simulink model "Y3Tiltrotor_sim3_IINDI_case2"  (R2025a)
settings: Solver=ode4  StartTime=0.0  StopTime=80  FixedStep=uavParam.sampleTime  RelTol=1e-3
PreLoadFcn:
  | filepath  = fileparts(get_param(bdroot, 'FileName'))
  | cd(filepath);
InitFcn:
  | Init_sim_IINDI_case2;
values from neighbouring files (symbols this model uses):
  a_HOD_p = 5    [Init_sim_IINDI_case2.m]    (also in Init_sim_IINDI_case2_1.m)
  a_HOD_q = 5    [Init_sim_IINDI_case2.m]    (also in Init_sim_IINDI_case2_1.m = 25)
  a_HOD_r = 5    [Init_sim_IINDI_case2.m]    (also in Init_sim_IINDI_case2_1.m)
  a_HOD_u = 5    [Init_sim_IINDI_case2.m]    (also in Init_sim_IINDI_case2_1.m = 15)
  a_HOD_v = 2    [Init_sim_IINDI_case2.m]    (also in Init_sim_IINDI_case2_1.m)
  a_HOD_w = 30    [Init_sim_IINDI_case2.m]    (also in Init_sim_IINDI_case2_1.m = 10)
  control = struct    [Init_sim_IINDI_case2.m]    (also in Init_sim_IINDI_case2_1.m)
  env = struct    [InitData.m]
  flightState = struct    [Init_sim_IINDI_case2.m]    (also in Init_sim_IINDI_case2_1.m)
  FWSpeed0 = 15    [Init_sim_IINDI_case2.m]    (also in Init_sim_IINDI_case2_1.m)
  k_lpf_p = 50    [Init_sim_IINDI_case2.m]    (also in Init_sim_IINDI_case2_1.m)
  k_lpf_q = 80    [Init_sim_IINDI_case2.m]    (also in Init_sim_IINDI_case2_1.m = 150)
  k_lpf_r = 100    [Init_sim_IINDI_case2.m]    (also in Init_sim_IINDI_case2_1.m)
  k_lpf_u = 8    [Init_sim_IINDI_case2.m]    (also in Init_sim_IINDI_case2_1.m)
  k_lpf_v = 1.5    [Init_sim_IINDI_case2.m]    (also in Init_sim_IINDI_case2_1.m)
  k_lpf_w = 50    [Init_sim_IINDI_case2.m]    (also in Init_sim_IINDI_case2_1.m)
  k_p = 5    [Init_sim_IINDI_case2.m]    (also in Init_sim_IINDI_case2_1.m)
  k_q = 12    [Init_sim_IINDI_case2.m]    (also in Init_sim_IINDI_case2_1.m)
  k_r = 0.1    [Init_sim_IINDI_case2.m]    (also in Init_sim_IINDI_case2_1.m)
  k_u = 0.2    [Init_sim_IINDI_case2.m]    (also in Init_sim_IINDI_case2_1.m = 1)
  k_v = 0.7    [Init_sim_IINDI_case2.m]    (also in Init_sim_IINDI_case2_1.m = 0.2)
  k_w = 2    [Init_sim_IINDI_case2.m]    (also in Init_sim_IINDI_case2_1.m)
  l_p = 30    [Init_sim_IINDI_case2.m]    (also in Init_sim_IINDI_case2_1.m)
  l_q = 15    [Init_sim_IINDI_case2.m]    (also in Init_sim_IINDI_case2_1.m)
  l_r = 25    [Init_sim_IINDI_case2.m]    (also in Init_sim_IINDI_case2_1.m)
  l_u = 1    [Init_sim_IINDI_case2.m]    (also in Init_sim_IINDI_case2_1.m = 0.8)
  l_v = 1.2    [Init_sim_IINDI_case2.m]    (also in Init_sim_IINDI_case2_1.m)
  l_w = 1    [Init_sim_IINDI_case2.m]    (also in Init_sim_IINDI_case2_1.m)
  lamda_p = 10    [Init_sim_IINDI_case2.m]    (also in Init_sim_IINDI_case2_1.m)
  lamda_q = 5    [Init_sim_IINDI_case2.m]    (also in Init_sim_IINDI_case2_1.m)
  lamda_r = 1    [Init_sim_IINDI_case2.m]    (also in Init_sim_IINDI_case2_1.m)
  lamda_u = 1    [Init_sim_IINDI_case2.m]    (also in Init_sim_IINDI_case2_1.m)
  lamda_v = 0.15    [Init_sim_IINDI_case2.m]    (also in Init_sim_IINDI_case2_1.m)
  lamda_w = 1    [Init_sim_IINDI_case2.m]    (also in Init_sim_IINDI_case2_1.m)
  uavParam = struct    [InitData.m]
undefined symbols (not defined in the file or in its folder): a_HOD, a_HOD_uvw, ControlSampleTime, F, Light, MIL, Newton, Raphson
libraries: slpidlib x30, SignalEditorBlockLib x15, simulink x3, aerolibtransform2 x3, sharedtransform x3, robotcorelib x3, matrix_library x3, aerolibasang x2, aerolibutil x2, aerolibwind2 x2, shared6dof x1, aerolibatmos2 x1
(part 6 of 7)

== system Y3Tiltrotor_sim3_IINDI_case2/Subsystem/多旋翼模态/Multirotor altitude control/Subsystem/Subsystem ==
  z_ref : Inport
  z : Inport  Port=2
  Action Port : ActionPort  ActionPortLabel=case [ 0 ]:
  Derivative : Derivative
  PID Controller : slpidlib/PID Controller  Controller=PID  Form=Parallel  TimeDomain=Continuous-time  UseExternalTs=off  SampleTime=ControlSampleTime  IntegratorMethod=Forward Euler  FilterMethod=Forward Euler  ControllerParametersSource=internal  P=control.MR.alt_P  I=control.MR.alt_I  UseKiTs=off  D=control.MR.alt_D  UseExternalDerivativeSource=off  N=100  UseFilter=on  TunerSelectOption=Transfer Function Based (PID Tuner App)  InitialConditionSource=internal  InitialConditionForIntegrator=0  InitialConditionForFilter=0  DifferentiatorICPrevScaledInput=0  ExternalReset=none  TrackingMode=off  Kt=1  LimitOutput=off  SatLimitsSource=internal  UpperSaturationLimit=control.maxMRvelocity  LowerSaturationLimit=-control.maxMRvelocity  LinearizeAsGain=on  AntiWindupMode=clamping  Kb=1  LimitIntegrator=off  UpperIntegratorSaturationLimit=inf  LowerIntegratorSaturationLimit=-inf  POutMin=[]  POutMax=[]  IOutMin=[]  IOutMax=[]  DOutMin=[]  DOutMax=[]  NOutMin=[]  NOutMax=[]  SumOutMin=[]  SumOutMax=[]  SaturationOutMin=[]  SaturationOutMax=[]  PParamMin=[]  PParamMax=[]  IParamMin=[]  IParamMax=[]  DParamMin=[]  DParamMax=[]  NParamMin=[]  NParamMax=[]  KbParamMin=[]  KbParamMax=[]  KtParamMin=[]  KtParamMax=[]  KbOutMin=[]  KbOutMax=[]  KtOutMin=[]  KtOutMax=[]  IntegratorOutMin=[]  IntegratorOutMax=[]  FilterOutMin=[]  FilterOutMax=[]  SumI1OutMin=[]  SumI1OutMax=[]  SumI2OutMin=[]  SumI2OutMax=[]  SumI3OutMin=[]  SumI3OutMax=[]  SumI4OutMin=[]  SumI4OutMax=[]  SumDOutMin=[]  SumDOutMax=[]  DifferentiatorOutMin=[]  DifferentiatorOutMax=[]  FilterDiffOutCoefMin=[]  FilterDiffOutCoefMax=[]  ReciprocalOutMin=[]  ReciprocalOutMax=[]  SumDenOutMin=[]  SumDenOutMax=[]  SumNumOutMin=[]  SumNumOutMax=[]  DivideOutMin=[]  DivideOutMax=[]  UdiffTsProdOutMin=[]  UdiffTsProdOutMax=[]  NTsProdOutMin=[]  NTsProdOutMax=[]  UintegralTsProdOutMin=[]  UintegralTsProdOutMax=[]  UngainTsProdOutMin=[]  UngainTsProdOutMax=[]  ClampingZeroOutDataTypeStr=Inherit: Inherit via back propagation  ClampingZeroOutMin=[]  ClampingZeroOutMax=[]  FilterDenConstantOutDataTypeStr=Inherit: Inherit via back propagation  FilterDenConstantOutMin=[]  FilterDenConstantOutMax=[]  PCopyOutDataTypeStr=Inherit: Inherit via back propagation  PCopyOutMin=[]  PCopyOutMax=[]  NCopyOutDataTypeStr=Inherit: Inherit via back propagation  NCopyOutMin=[]  NCopyOutMax=[]  IntegratorContinuousStateAttributes=''  IntegratorStateMustResolveToSignalObject=off  IntegratorRTWStateStorageClass=Auto  FilterContinuousStateAttributes=''  FilterStateMustResolveToSignalObject=off  FilterRTWStateStorageClass=Auto  ParallelPVariant=InternalParameters  IdealPVariant=Disabled  IVariant=InternalParameters  DVariant=InternalParameters  IntegratorVariant=Continuous  SatVariant=Disabled  AWVariant=Passthrough  PCopyVariant=Disabled  TRVariant=Disabled  FdbkBlocksVariant=Forward  IdealPFdbkVariant=Disabled  SatFdbkVariant=Disabled  DerivativeFilterVariant=ContFilter  NVariant=InternalParameters  NCopyVariant=Disabled  FilterICVariant=InternalICsFilter  IntegratorICVariant=InternalICs  ExternalResetVariant=Disabled  TRSumVariant=Passthrough  SumFdbkVariant=Disabled  SumVariant=Sum_PID  TsampFilterVariant=InternalTs  TsampNgainVariant=Passthrough  TsampIntegralVariant=Disabled_SignalSpec  ExternalSaturationOutDataTypeStr=Inherit: Same as second input  DerivativeSourceVariant=ErrorSignal  PreIntVariant=InternalPreInt
  Saturation : Saturate  UpperLimit=control.maxMRvelocity  LowerLimit=-control.maxMRvelocity
  Sum : Sum  Inputs=|+-
  Sum1 : Sum  Inputs=++|
  Transfer Fcn1 : TransferFcn  Numerator=[5]  Denominator=[1 5]
  Transfer Fcn7 : TransferFcn  Numerator=[10]  Denominator=[1 10]
  PID_vz_cmd : Outport
  wires:
  z_ref/1 -> Transfer Fcn1/1
  z/1 -> Sum/2
  Sum/1 -> PID Controller/1  "e_z_IINDI"
  PID Controller/1 -> Sum1/2
  Derivative/1 -> Transfer Fcn7/1
  Sum1/1 -> Saturation/1
  Saturation/1 -> PID_vz_cmd/1
  Transfer Fcn7/1 -> Sum1/1
  Transfer Fcn1/1 -> Derivative/1, Sum/1  "z_ref"

== system Y3Tiltrotor_sim3_IINDI_case2/Subsystem/多旋翼模态/Multirotor attitude control (IINDI)/INDI in vector form/Subsystem ==
  original : Inport
  Demux : Demux  Outputs=3
  Mux : Mux  Inputs=3
  Transfer Fcn1 : TransferFcn  Numerator=[k_lpf_q]  Denominator=[1 k_lpf_q]
  Transfer Fcn2 : TransferFcn  Numerator=[k_lpf_r]  Denominator=[1 k_lpf_r]
  Transfer Fcn3 : TransferFcn  Numerator=[k_lpf_p]  Denominator=[1 k_lpf_p]
  LPF : Outport
  wires:
  Demux/2 -> Transfer Fcn1/1
  Demux/1 -> Transfer Fcn3/1
  Mux/1 -> LPF/1
  Transfer Fcn3/1 -> Mux/1
  Transfer Fcn1/1 -> Mux/2
  Transfer Fcn2/1 -> Mux/3
  Demux/3 -> Transfer Fcn2/1
  original/1 -> Demux/1

== system Y3Tiltrotor_sim3_IINDI_case2/Subsystem/多旋翼模态/Multirotor attitude control (IINDI)/INDI in vector form/Subsystem1 ==
  original : Inport
  Demux : Demux  Outputs=3
  Mux : Mux  Inputs=3
  Transfer Fcn1 : TransferFcn  Numerator=[k_lpf_q]  Denominator=[1 k_lpf_q]
  Transfer Fcn2 : TransferFcn  Numerator=[k_lpf_r]  Denominator=[1 k_lpf_r]
  Transfer Fcn3 : TransferFcn  Numerator=[k_lpf_p]  Denominator=[1 k_lpf_p]
  LPF : Outport
  wires:
  Demux/2 -> Transfer Fcn1/1
  Demux/1 -> Transfer Fcn3/1
  Mux/1 -> LPF/1
  Transfer Fcn3/1 -> Mux/1
  Transfer Fcn1/1 -> Mux/2
  Transfer Fcn2/1 -> Mux/3
  Demux/3 -> Transfer Fcn2/1
  original/1 -> Demux/1

== system Y3Tiltrotor_sim3_IINDI_case2/Subsystem/多旋翼模态/Multirotor attitude control (IINDI)/INDI in vector form/Subsystem2 ==
  original : Inport
  Demux : Demux  Outputs=3
  Mux : Mux  Inputs=3
  Transfer Fcn1 : TransferFcn  Numerator=[k_lpf_q]  Denominator=[1 k_lpf_q]
  Transfer Fcn2 : TransferFcn  Numerator=[k_lpf_r]  Denominator=[1 k_lpf_r]
  Transfer Fcn3 : TransferFcn  Numerator=[k_lpf_p]  Denominator=[1 k_lpf_p]
  LPF : Outport
  wires:
  Demux/2 -> Transfer Fcn1/1
  Demux/1 -> Transfer Fcn3/1
  Mux/1 -> LPF/1
  Transfer Fcn3/1 -> Mux/1
  Transfer Fcn1/1 -> Mux/2
  Transfer Fcn2/1 -> Mux/3
  Demux/3 -> Transfer Fcn2/1
  original/1 -> Demux/1

== system Y3Tiltrotor_sim3_IINDI_case2/Subsystem/多旋翼模态/Multirotor attitude control (IINDI)/Improved INDI in vector form/6阶HOD ==
  X1 : Inport
  Gain : Gain  Gain=[4*a_HOD_p^2 0 0;0 4*a_HOD_q^2 0;0 0 4*a_HOD_r^2]  Multiplication=Matrix(K*u) (u vector)
  Gain1 : Gain  Gain=[4*a_HOD_p 0 0;0 4*a_HOD_q 0;0 0 4*a_HOD_r]  Multiplication=Matrix(K*u) (u vector)
  Integrator : Integrator  InitialCondition=[0 0 0]'
  Integrator1 : Integrator  InitialCondition=[0 0 0]'
  Sum : Sum  Inputs=|+-
  Sum1 : Sum  Inputs=++|
  X1_dot_hat : Outport
  wires:
  Gain1/1 -> Sum1/1
  Integrator1/1 -> Sum1/2  "x2_hat"
  Gain/1 -> Integrator1/1
  Sum1/1 -> Integrator/1, X1_dot_hat/1
  Sum/1 -> Gain1/1, Gain/1
  X1/1 -> Sum/1
  Integrator/1 -> Sum/2  "x1_hat"

== system Y3Tiltrotor_sim3_IINDI_case2/Subsystem/多旋翼模态/Multirotor attitude control (IINDI)/Improved INDI in vector form/6阶HOD1 ==
  X1 : Inport
  Gain : Gain  Gain=[4*a_HOD_p^2 0 0;0 4*a_HOD_q^2 0;0 0 4*a_HOD_r^2]  Multiplication=Matrix(K*u) (u vector)
  Gain1 : Gain  Gain=[4*a_HOD_p 0 0;0 4*a_HOD_q 0;0 0 4*a_HOD_r]  Multiplication=Matrix(K*u) (u vector)
  Integrator : Integrator  InitialCondition=[0 0 0]'
  Integrator1 : Integrator  InitialCondition=[0 0 0]'
  Sum : Sum  Inputs=|+-
  Sum1 : Sum  Inputs=++|
  X1_dot_hat : Outport
  wires:
  Integrator/1 -> Sum/2  "x1_hat"
  X1/1 -> Sum/1
  Sum/1 -> Gain/1, Gain1/1
  Sum1/1 -> X1_dot_hat/1, Integrator/1
  Gain/1 -> Integrator1/1
  Integrator1/1 -> Sum1/2  "x2_hat"
  Gain1/1 -> Sum1/1

== system Y3Tiltrotor_sim3_IINDI_case2/Subsystem/多旋翼模态/Multirotor attitude control (IINDI)/Improved INDI in vector form/CFO ==
  x1_dot : Inport
  x1 : Inport  Port=2
  bu : Inport  Port=3
  Gain : Gain  Gain=[l_p 0 0;0 l_q 0;0 0 l_r]  Multiplication=Matrix(K*u) (u vector)
  Gain1 : Gain  Gain=[lamda_p 0 0;0 lamda_q 0;0 0 lamda_r]  Multiplication=Matrix(K*u) (u vector)
  Integrator : Integrator  InitialCondition=[0 0 0]'
  Integrator1 : Integrator  InitialCondition=[0 0 0]'
  Sum : Sum  Inputs=|+-
  Sum1 : Sum  Inputs=+++
  Sum2 : Sum  Inputs=++|
  d_hat : Outport
  wires:
  Sum2/1 -> d_hat/1, Sum1/1
  Integrator1/1 -> Sum2/2  "x2_hat"
  Gain1/1 -> Integrator1/1
  Sum/1 -> Gain/1
  Gain/1 -> Gain1/1, Sum2/1
  bu/1 -> Sum1/3
  x1_dot/1 -> Sum1/2
  Sum1/1 -> Integrator/1
  Integrator/1 -> Sum/2  "x1_hat"
  x1/1 -> Sum/1

== system Y3Tiltrotor_sim3_IINDI_case2/Subsystem/多旋翼模态/Multirotor attitude control (IINDI)/Improved INDI in vector form/Subsystem ==
  original : Inport
  Demux : Demux  Outputs=3
  Mux : Mux  Inputs=3
  Transfer Fcn1 : TransferFcn  Numerator=[k_lpf_q]  Denominator=[1 k_lpf_q]
  Transfer Fcn2 : TransferFcn  Numerator=[k_lpf_r]  Denominator=[1 k_lpf_r]
  Transfer Fcn3 : TransferFcn  Numerator=[k_lpf_p]  Denominator=[1 k_lpf_p]
  LPF : Outport
  wires:
  Demux/2 -> Transfer Fcn1/1
  Demux/1 -> Transfer Fcn3/1
  Mux/1 -> LPF/1
  Transfer Fcn3/1 -> Mux/1
  Transfer Fcn1/1 -> Mux/2
  Transfer Fcn2/1 -> Mux/3
  Demux/3 -> Transfer Fcn2/1
  original/1 -> Demux/1

== system Y3Tiltrotor_sim3_IINDI_case2/Subsystem/多旋翼模态/Multirotor attitude control (IINDI)/Improved INDI in vector form/Subsystem2 ==
  original : Inport
  Demux : Demux  Outputs=3
  Mux : Mux  Inputs=3
  Transfer Fcn1 : TransferFcn  Numerator=[k_lpf_q]  Denominator=[1 k_lpf_q]
  Transfer Fcn2 : TransferFcn  Numerator=[k_lpf_r]  Denominator=[1 k_lpf_r]
  Transfer Fcn3 : TransferFcn  Numerator=[k_lpf_p]  Denominator=[1 k_lpf_p]
  LPF : Outport
  wires:
  Demux/2 -> Transfer Fcn1/1
  Demux/1 -> Transfer Fcn3/1
  Mux/1 -> LPF/1
  Transfer Fcn3/1 -> Mux/1
  Transfer Fcn1/1 -> Mux/2
  Transfer Fcn2/1 -> Mux/3
  Demux/3 -> Transfer Fcn2/1
  original/1 -> Demux/1

== system Y3Tiltrotor_sim3_IINDI_case2/Subsystem/多旋翼模态/Multirotor attitude control (IINDI)/Improved INDI_p/2阶HOD ==
  X1 : Inport
  Gain : Gain  Gain=4*a_HOD^2
  Gain1 : Gain  Gain=4*a_HOD
  Integrator : Integrator
  Integrator1 : Integrator
  Sum : Sum  Inputs=|+-
  Sum1 : Sum  Inputs=++|
  X1_dot_hat : Outport
  wires:
  Gain1/1 -> Sum1/1
  Integrator1/1 -> Sum1/2  "x2_hat"
  Gain/1 -> Integrator1/1
  Sum1/1 -> Integrator/1, X1_dot_hat/1
  Sum/1 -> Gain1/1, Gain/1
  X1/1 -> Sum/1
  Integrator/1 -> Sum/2  "x1_hat"

== system Y3Tiltrotor_sim3_IINDI_case2/Subsystem/多旋翼模态/Multirotor attitude control (IINDI)/Improved INDI_p/CFO ==
  x1_dot : Inport
  x1 : Inport  Port=2
  bu : Inport  Port=3
  Gain : Gain  Gain=l_p
  Gain1 : Gain  Gain=lamda_p
  Integrator : Integrator
  Integrator1 : Integrator
  Sum : Sum  Inputs=|+-
  Sum1 : Sum  Inputs=+++
  Sum2 : Sum  Inputs=++|
  d_hat : Outport
  wires:
  Sum2/1 -> d_hat/1, Sum1/1
  Integrator1/1 -> Sum2/2  "x2_hat"
  Gain1/1 -> Integrator1/1
  Sum/1 -> Gain/1
  Gain/1 -> Gain1/1, Sum2/1
  bu/1 -> Sum1/3
  x1_dot/1 -> Sum1/2
  Sum1/1 -> Integrator/1
  Integrator/1 -> Sum/2  "x1_hat"
  x1/1 -> Sum/1

== system Y3Tiltrotor_sim3_IINDI_case2/Subsystem/多旋翼模态/Multirotor attitude control (IINDI)/Improved INDI_q/2阶HOD ==
  X1 : Inport
  Gain : Gain  Gain=4*a_HOD^2
  Gain1 : Gain  Gain=4*a_HOD
  Integrator : Integrator
  Integrator1 : Integrator
  Sum : Sum  Inputs=|+-
  Sum1 : Sum  Inputs=++|
  X1_dot_hat : Outport
  wires:
  Integrator/1 -> Sum/2  "x1_hat"
  X1/1 -> Sum/1
  Sum/1 -> Gain/1, Gain1/1
  Sum1/1 -> X1_dot_hat/1, Integrator/1
  Gain/1 -> Integrator1/1
  Integrator1/1 -> Sum1/2  "x2_hat"
  Gain1/1 -> Sum1/1

== system Y3Tiltrotor_sim3_IINDI_case2/Subsystem/多旋翼模态/Multirotor attitude control (IINDI)/Improved INDI_q/CFO ==
  x1_dot : Inport
  x1 : Inport  Port=2
  bu : Inport  Port=3
  Gain : Gain  Gain=l_q
  Gain1 : Gain  Gain=lamda_q
  Integrator : Integrator
  Integrator1 : Integrator
  Sum : Sum  Inputs=|+-
  Sum1 : Sum  Inputs=+++
  Sum2 : Sum  Inputs=++|
  d_hat : Outport
  wires:
  x1/1 -> Sum/1
  Integrator/1 -> Sum/2  "x1_hat"
  Sum1/1 -> Integrator/1
  x1_dot/1 -> Sum1/2
  bu/1 -> Sum1/3
  Gain/1 -> Sum2/1, Gain1/1
  Sum/1 -> Gain/1
  Gain1/1 -> Integrator1/1
  Integrator1/1 -> Sum2/2  "x2_hat"
  Sum2/1 -> Sum1/1, d_hat/1

== system Y3Tiltrotor_sim3_IINDI_case2/Subsystem/多旋翼模态/Multirotor attitude control (IINDI)/Improved INDI_r/2阶HOD ==
  X1 : Inport
  Gain : Gain  Gain=4*a_HOD^2
  Gain1 : Gain  Gain=4*a_HOD
  Integrator : Integrator
  Integrator1 : Integrator
  Sum : Sum  Inputs=|+-
  Sum1 : Sum  Inputs=++|
  X1_dot_hat : Outport
  wires:
  Gain1/1 -> Sum1/1
  Integrator1/1 -> Sum1/2  "x2_hat"
  Gain/1 -> Integrator1/1
  Sum1/1 -> Integrator/1, X1_dot_hat/1
  Sum/1 -> Gain1/1, Gain/1
  X1/1 -> Sum/1
  Integrator/1 -> Sum/2  "x1_hat"

== system Y3Tiltrotor_sim3_IINDI_case2/Subsystem/多旋翼模态/Multirotor attitude control (IINDI)/Improved INDI_r/CFO ==
  x1_dot : Inport
  x1 : Inport  Port=2
  bu : Inport  Port=3
  Gain : Gain  Gain=l_r
  Gain1 : Gain  Gain=lamda_r
  Integrator : Integrator
  Integrator1 : Integrator
  Sum : Sum  Inputs=|+-
  Sum1 : Sum  Inputs=+++
  Sum2 : Sum  Inputs=++|
  d_hat : Outport
  wires:
  Sum2/1 -> d_hat/1, Sum1/1
  Integrator1/1 -> Sum2/2  "x2_hat"
  Gain1/1 -> Integrator1/1
  Sum/1 -> Gain/1
  Gain/1 -> Gain1/1, Sum2/1
  bu/1 -> Sum1/3
  x1_dot/1 -> Sum1/2
  Sum1/1 -> Integrator/1
  Integrator/1 -> Sum/2  "x1_hat"
  x1/1 -> Sum/1

== system Y3Tiltrotor_sim3_IINDI_case2/Subsystem/多旋翼模态/Multirotor attitude control (IINDI)/Subsystem/Subsystem ==
  Euler_d : Inport
  Euler : Inport  Port=2
  Action Port : ActionPort  ActionPortLabel=case [ 0 ]:
  Gain1 : Gain  Gain=pi/180
  PID Controller4 : slpidlib/PID Controller  Controller=PI  Form=Parallel  TimeDomain=Continuous-time  UseExternalTs=off  SampleTime=ControlSampleTime  IntegratorMethod=Forward Euler  FilterMethod=Forward Euler  ControllerParametersSource=internal  P=control.MR.yaw_P  I=control.MR.yaw_I  UseKiTs=off  D=0  UseExternalDerivativeSource=off  N=100  UseFilter=on  TunerSelectOption=Transfer Function Based (PID Tuner App)  InitialConditionSource=internal  InitialConditionForIntegrator=0  InitialConditionForFilter=0  DifferentiatorICPrevScaledInput=0  ExternalReset=none  TrackingMode=off  Kt=1  LimitOutput=on  SatLimitsSource=internal  UpperSaturationLimit=control.maxRollRate  LowerSaturationLimit=control.minRollRate  LinearizeAsGain=on  AntiWindupMode=clamping  Kb=1  LimitIntegrator=off  UpperIntegratorSaturationLimit=inf  LowerIntegratorSaturationLimit=-inf  POutMin=[]  POutMax=[]  IOutMin=[]  IOutMax=[]  DOutMin=[]  DOutMax=[]  NOutMin=[]  NOutMax=[]  SumOutMin=[]  SumOutMax=[]  SaturationOutMin=[]  SaturationOutMax=[]  PParamMin=[]  PParamMax=[]  IParamMin=[]  IParamMax=[]  DParamMin=[]  DParamMax=[]  NParamMin=[]  NParamMax=[]  KbParamMin=[]  KbParamMax=[]  KtParamMin=[]  KtParamMax=[]  KbOutMin=[]  KbOutMax=[]  KtOutMin=[]  KtOutMax=[]  IntegratorOutMin=[]  IntegratorOutMax=[]  FilterOutMin=[]  FilterOutMax=[]  SumI1OutMin=[]  SumI1OutMax=[]  SumI2OutMin=[]  SumI2OutMax=[]  SumI3OutMin=[]  SumI3OutMax=[]  SumI4OutMin=[]  SumI4OutMax=[]  SumDOutMin=[]  SumDOutMax=[]  DifferentiatorOutMin=[]  DifferentiatorOutMax=[]  FilterDiffOutCoefMin=[]  FilterDiffOutCoefMax=[]  ReciprocalOutMin=[]  ReciprocalOutMax=[]  SumDenOutMin=[]  SumDenOutMax=[]  SumNumOutMin=[]  SumNumOutMax=[]  DivideOutMin=[]  DivideOutMax=[]  UdiffTsProdOutMin=[]  UdiffTsProdOutMax=[]  NTsProdOutMin=[]  NTsProdOutMax=[]  UintegralTsProdOutMin=[]  UintegralTsProdOutMax=[]  UngainTsProdOutMin=[]  UngainTsProdOutMax=[]  ClampingZeroOutDataTypeStr=Inherit: Inherit via back propagation  ClampingZeroOutMin=[]  ClampingZeroOutMax=[]  FilterDenConstantOutDataTypeStr=Inherit: Inherit via back propagation  FilterDenConstantOutMin=[]  FilterDenConstantOutMax=[]  PCopyOutDataTypeStr=Inherit: Inherit via back propagation  PCopyOutMin=[]  PCopyOutMax=[]  NCopyOutDataTypeStr=Inherit: Inherit via back propagation  NCopyOutMin=[]  NCopyOutMax=[]  IntegratorContinuousStateAttributes=''  IntegratorStateMustResolveToSignalObject=off  IntegratorRTWStateStorageClass=Auto  FilterContinuousStateAttributes=''  FilterStateMustResolveToSignalObject=off  FilterRTWStateStorageClass=Auto  ParallelPVariant=InternalParameters  IdealPVariant=Disabled  IVariant=InternalParameters  DVariant=Disabled  IntegratorVariant=Continuous  SatVariant=Enabled  AWVariant=ContClampingParallel  PCopyVariant=Disabled  TRVariant=Disabled  FdbkBlocksVariant=Forward  IdealPFdbkVariant=Disabled  SatFdbkVariant=Disabled  DerivativeFilterVariant=Disabled  NVariant=Disabled  NCopyVariant=Disabled_SignalSpec  FilterICVariant=Disabled  IntegratorICVariant=InternalICs  ExternalResetVariant=Disabled  TRSumVariant=Passthrough  SumFdbkVariant=Disabled  SumVariant=Sum_PI  TsampFilterVariant=InternalTs  TsampNgainVariant=Passthrough  TsampIntegralVariant=Disabled_SignalSpec  ExternalSaturationOutDataTypeStr=Inherit: Same as second input  DerivativeSourceVariant=Disabled  PreIntVariant=InternalPreInt
  Selector4 : Selector  InputPortWidth=3  IndexOptions=Index vector (dialog)  Indices=3  OutputSizes=1
  Selector8 : Selector  InputPortWidth=3  IndexOptions=Index vector (dialog)  Indices=3  OutputSizes=1
  Sum4 : Sum  Inputs=|+-
  Transfer Fcn2 : TransferFcn  Numerator=[5]  Denominator=[1 5]
  MR_r_d : Outport
  wires:
  Euler/1 -> Selector8/1
  Gain1/1 -> Transfer Fcn2/1
  Selector4/1 -> Gain1/1
  Transfer Fcn2/1 -> Sum4/1
  Selector8/1 -> Sum4/2
  PID Controller4/1 -> MR_r_d/1
  Sum4/1 -> PID Controller4/1  "e_yaw_IINDI"
  Euler_d/1 -> Selector4/1

== system Y3Tiltrotor_sim3_IINDI_case2/Subsystem/多旋翼模态/Multirotor attitude control (IINDI)/Subsystem/Subsystem1 ==
  note: 遥控器在中位时，偏航角保持
  YawRate_d : Inport
  Yaw : Inport  Port=2
  YawRate : Inport  Port=3
  Action Port : ActionPort  ActionPortLabel=case [ 1 ]:
  MATLAB Function : MATLAB Function
  PID Controller4 : slpidlib/PID Controller  Controller=PI  Form=Parallel  TimeDomain=Continuous-time  UseExternalTs=off  SampleTime=ControlSampleTime  IntegratorMethod=Forward Euler  FilterMethod=Forward Euler  ControllerParametersSource=internal  P=control.MR.yaw_P  I=control.MR.yaw_I  UseKiTs=off  D=0  UseExternalDerivativeSource=off  N=100  UseFilter=on  TunerSelectOption=Transfer Function Based (PID Tuner App)  InitialConditionSource=internal  InitialConditionForIntegrator=0  InitialConditionForFilter=0  DifferentiatorICPrevScaledInput=0  ExternalReset=none  TrackingMode=off  Kt=1  LimitOutput=on  SatLimitsSource=internal  UpperSaturationLimit=control.maxRollRate  LowerSaturationLimit=control.minRollRate  LinearizeAsGain=on  AntiWindupMode=clamping  Kb=1  LimitIntegrator=off  UpperIntegratorSaturationLimit=inf  LowerIntegratorSaturationLimit=-inf  POutMin=[]  POutMax=[]  IOutMin=[]  IOutMax=[]  DOutMin=[]  DOutMax=[]  NOutMin=[]  NOutMax=[]  SumOutMin=[]  SumOutMax=[]  SaturationOutMin=[]  SaturationOutMax=[]  PParamMin=[]  PParamMax=[]  IParamMin=[]  IParamMax=[]  DParamMin=[]  DParamMax=[]  NParamMin=[]  NParamMax=[]  KbParamMin=[]  KbParamMax=[]  KtParamMin=[]  KtParamMax=[]  KbOutMin=[]  KbOutMax=[]  KtOutMin=[]  KtOutMax=[]  IntegratorOutMin=[]  IntegratorOutMax=[]  FilterOutMin=[]  FilterOutMax=[]  SumI1OutMin=[]  SumI1OutMax=[]  SumI2OutMin=[]  SumI2OutMax=[]  SumI3OutMin=[]  SumI3OutMax=[]  SumI4OutMin=[]  SumI4OutMax=[]  SumDOutMin=[]  SumDOutMax=[]  DifferentiatorOutMin=[]  DifferentiatorOutMax=[]  FilterDiffOutCoefMin=[]  FilterDiffOutCoefMax=[]  ReciprocalOutMin=[]  ReciprocalOutMax=[]  SumDenOutMin=[]  SumDenOutMax=[]  SumNumOutMin=[]  SumNumOutMax=[]  DivideOutMin=[]  DivideOutMax=[]  UdiffTsProdOutMin=[]  UdiffTsProdOutMax=[]  NTsProdOutMin=[]  NTsProdOutMax=[]  UintegralTsProdOutMin=[]  UintegralTsProdOutMax=[]  UngainTsProdOutMin=[]  UngainTsProdOutMax=[]  ClampingZeroOutDataTypeStr=Inherit: Inherit via back propagation  ClampingZeroOutMin=[]  ClampingZeroOutMax=[]  FilterDenConstantOutDataTypeStr=Inherit: Inherit via back propagation  FilterDenConstantOutMin=[]  FilterDenConstantOutMax=[]  PCopyOutDataTypeStr=Inherit: Inherit via back propagation  PCopyOutMin=[]  PCopyOutMax=[]  NCopyOutDataTypeStr=Inherit: Inherit via back propagation  NCopyOutMin=[]  NCopyOutMax=[]  IntegratorContinuousStateAttributes=''  IntegratorStateMustResolveToSignalObject=off  IntegratorRTWStateStorageClass=Auto  FilterContinuousStateAttributes=''  FilterStateMustResolveToSignalObject=off  FilterRTWStateStorageClass=Auto  ParallelPVariant=InternalParameters  IdealPVariant=Disabled  IVariant=InternalParameters  DVariant=Disabled  IntegratorVariant=Continuous  SatVariant=Enabled  AWVariant=ContClampingParallel  PCopyVariant=Disabled  TRVariant=Disabled  FdbkBlocksVariant=Forward  IdealPFdbkVariant=Disabled  SatFdbkVariant=Disabled  DerivativeFilterVariant=Disabled  NVariant=Disabled  NCopyVariant=Disabled_SignalSpec  FilterICVariant=Disabled  IntegratorICVariant=InternalICs  ExternalResetVariant=Disabled  TRSumVariant=Passthrough  SumFdbkVariant=Disabled  SumVariant=Sum_PI  TsampFilterVariant=InternalTs  TsampNgainVariant=Passthrough  TsampIntegralVariant=Disabled_SignalSpec  ExternalSaturationOutDataTypeStr=Inherit: Same as second input  DerivativeSourceVariant=Disabled  PreIntVariant=InternalPreInt
  Sum1 : Sum  Inputs=|++
  Sum4 : Sum  Inputs=|+-
  r_d : Outport
  wires:
  Yaw/1 -> MATLAB Function/2(yaw), Sum4/2
  PID Controller4/1 -> Sum1/2
  Sum4/1 -> PID Controller4/1
  YawRate/1 -> MATLAB Function/3(yaw_rate)
  MATLAB Function/2(yaw_d) -> Sum4/1
  MATLAB Function/1(yaw_rate_d) -> Sum1/1
  YawRate_d/1 -> MATLAB Function/1(yaw_rate_desired)
  Sum1/1 -> r_d/1

== system Y3Tiltrotor_sim3_IINDI_case2/Subsystem/多旋翼模态/Velocity Control/IINDI_u/2阶HOD ==
  X1 : Inport
  Gain : Gain  Gain=4*a_HOD_u^2
  Gain1 : Gain  Gain=4*a_HOD_u
  Integrator : Integrator
  Integrator1 : Integrator
  Sum : Sum  Inputs=|+-
  Sum1 : Sum  Inputs=++|
  X1_dot_hat : Outport
  wires:
  Gain1/1 -> Sum1/1
  Integrator1/1 -> Sum1/2  "x2_hat"
  Gain/1 -> Integrator1/1
  Sum1/1 -> Integrator/1, X1_dot_hat/1
  Sum/1 -> Gain1/1, Gain/1
  X1/1 -> Sum/1
  Integrator/1 -> Sum/2  "x1_hat"

== system Y3Tiltrotor_sim3_IINDI_case2/Subsystem/多旋翼模态/Velocity Control/IINDI_u/2阶HOD1 ==
  X1 : Inport
  Gain : Gain  Gain=4*a_HOD_u^2
  Gain1 : Gain  Gain=4*a_HOD_u
  Integrator : Integrator
  Integrator1 : Integrator
  Sum : Sum  Inputs=|+-
  Sum1 : Sum  Inputs=++|
  X1_dot_hat : Outport
  wires:
  Integrator/1 -> Sum/2  "x1_hat"
  X1/1 -> Sum/1
  Sum/1 -> Gain/1, Gain1/1
  Sum1/1 -> X1_dot_hat/1, Integrator/1
  Gain/1 -> Integrator1/1
  Integrator1/1 -> Sum1/2  "x2_hat"
  Gain1/1 -> Sum1/1

== system Y3Tiltrotor_sim3_IINDI_case2/Subsystem/多旋翼模态/Velocity Control/IINDI_u/CFO ==
  x1_dot : Inport
  x1 : Inport  Port=2
  bu : Inport  Port=3
  Gain : Gain  Gain=l_u
  Gain1 : Gain  Gain=lamda_u
  Integrator : Integrator
  Integrator1 : Integrator
  Sum : Sum  Inputs=|+-
  Sum1 : Sum  Inputs=+++
  Sum2 : Sum  Inputs=++|
  d_hat : Outport
  wires:
  Sum2/1 -> d_hat/1, Sum1/1
  Integrator1/1 -> Sum2/2  "x2_hat"
  Gain1/1 -> Integrator1/1
  Sum/1 -> Gain/1
  Gain/1 -> Gain1/1, Sum2/1
  bu/1 -> Sum1/3
  x1_dot/1 -> Sum1/2
  Sum1/1 -> Integrator/1
  Integrator/1 -> Sum/2  "x1_hat"
  x1/1 -> Sum/1

== system Y3Tiltrotor_sim3_IINDI_case2/Subsystem/多旋翼模态/Velocity Control/IINDI_v/2阶HOD ==
  X1 : Inport
  Gain : Gain  Gain=4*a_HOD_v^2
  Gain1 : Gain  Gain=4*a_HOD_v
  Integrator : Integrator
  Integrator1 : Integrator
  Sum : Sum  Inputs=|+-
  Sum1 : Sum  Inputs=++|
  X1_dot_hat : Outport
  wires:
  Gain1/1 -> Sum1/1
  Integrator1/1 -> Sum1/2  "x2_hat"
  Gain/1 -> Integrator1/1
  Sum1/1 -> Integrator/1, X1_dot_hat/1
  Sum/1 -> Gain1/1, Gain/1
  X1/1 -> Sum/1
  Integrator/1 -> Sum/2  "x1_hat"

== system Y3Tiltrotor_sim3_IINDI_case2/Subsystem/多旋翼模态/Velocity Control/IINDI_v/2阶HOD1 ==
  X1 : Inport
  Gain : Gain  Gain=4*a_HOD_v^2
  Gain1 : Gain  Gain=4*a_HOD_v
  Integrator : Integrator
  Integrator1 : Integrator
  Sum : Sum  Inputs=|+-
  Sum1 : Sum  Inputs=++|
  X1_dot_hat : Outport
  wires:
  Integrator/1 -> Sum/2  "x1_hat"
  X1/1 -> Sum/1
  Sum/1 -> Gain/1, Gain1/1
  Sum1/1 -> X1_dot_hat/1, Integrator/1
  Gain/1 -> Integrator1/1
  Integrator1/1 -> Sum1/2  "x2_hat"
  Gain1/1 -> Sum1/1

== system Y3Tiltrotor_sim3_IINDI_case2/Subsystem/多旋翼模态/Velocity Control/IINDI_v/CFO ==
  x1_dot : Inport
  x1 : Inport  Port=2
  bu : Inport  Port=3
  Gain : Gain  Gain=l_v
  Gain1 : Gain  Gain=lamda_v
  Integrator : Integrator
  Integrator1 : Integrator
  Sum : Sum  Inputs=|+-
  Sum1 : Sum  Inputs=+++
  Sum2 : Sum  Inputs=++|
  d_hat : Outport
  wires:
  Sum2/1 -> d_hat/1, Sum1/1
  Integrator1/1 -> Sum2/2  "x2_hat"
  Gain1/1 -> Integrator1/1
  Sum/1 -> Gain/1
  Gain/1 -> Gain1/1, Sum2/1
  bu/1 -> Sum1/3
  x1_dot/1 -> Sum1/2
  Sum1/1 -> Integrator/1
  Integrator/1 -> Sum/2  "x1_hat"
  x1/1 -> Sum/1

== system Y3Tiltrotor_sim3_IINDI_case2/Subsystem/多旋翼模态/Velocity Control/IINDI_v1/2阶HOD ==
  X1 : Inport
  Gain : Gain  Gain=4*a_HOD_v^2
  Gain1 : Gain  Gain=4*a_HOD_v
  Integrator : Integrator
  Integrator1 : Integrator
  Sum : Sum  Inputs=|+-
  Sum1 : Sum  Inputs=++|
  X1_dot_hat : Outport
  wires:
  Gain1/1 -> Sum1/1
  Integrator1/1 -> Sum1/2  "x2_hat"
  Gain/1 -> Integrator1/1
  Sum1/1 -> Integrator/1, X1_dot_hat/1
  Sum/1 -> Gain1/1, Gain/1
  X1/1 -> Sum/1
  Integrator/1 -> Sum/2  "x1_hat"

== system Y3Tiltrotor_sim3_IINDI_case2/Subsystem/多旋翼模态/Velocity Control/IINDI_v1/CFO ==
  x1_dot : Inport
  x1 : Inport  Port=2
  bu : Inport  Port=3
  Gain : Gain  Gain=l_v
  Gain1 : Gain  Gain=lamda_v
  Integrator : Integrator
  Integrator1 : Integrator
  Sum : Sum  Inputs=|+-
  Sum1 : Sum  Inputs=+++
  Sum2 : Sum  Inputs=++|
  d_hat : Outport
  wires:
  Sum2/1 -> d_hat/1, Sum1/1
  Integrator1/1 -> Sum2/2  "x2_hat"
  Gain1/1 -> Integrator1/1
  Sum/1 -> Gain/1
  Gain/1 -> Gain1/1, Sum2/1
  bu/1 -> Sum1/3
  x1_dot/1 -> Sum1/2
  Sum1/1 -> Integrator/1
  Integrator/1 -> Sum/2  "x1_hat"
  x1/1 -> Sum/1

== system Y3Tiltrotor_sim3_IINDI_case2/Subsystem/多旋翼模态/Velocity Control/IINDI_w/2阶HOD ==
  X1 : Inport
  Gain : Gain  Gain=4*a_HOD_w^2
  Gain1 : Gain  Gain=4*a_HOD_w
  Integrator : Integrator
  Integrator1 : Integrator
  Sum : Sum  Inputs=|+-
  Sum1 : Sum  Inputs=++|
  X1_dot_hat : Outport
  wires:
  Gain1/1 -> Sum1/1
  Integrator1/1 -> Sum1/2  "x2_hat"
  Gain/1 -> Integrator1/1
  Sum1/1 -> Integrator/1, X1_dot_hat/1
  Sum/1 -> Gain1/1, Gain/1
  X1/1 -> Sum/1
  Integrator/1 -> Sum/2  "x1_hat"

== system Y3Tiltrotor_sim3_IINDI_case2/Subsystem/多旋翼模态/Velocity Control/IINDI_w/CFO ==
  x1_dot : Inport
  x1 : Inport  Port=2
  bu : Inport  Port=3
  Gain : Gain  Gain=l_w
  Gain1 : Gain  Gain=lamda_w
  Integrator : Integrator
  Integrator1 : Integrator
  Sum : Sum  Inputs=|+-
  Sum1 : Sum  Inputs=+++
  Sum2 : Sum  Inputs=++|
  d_hat : Outport
  wires:
  Sum2/1 -> d_hat/1, Sum1/1
  Integrator1/1 -> Sum2/2  "x2_hat"
  Gain1/1 -> Integrator1/1
  Sum/1 -> Gain/1
  Gain/1 -> Gain1/1, Sum2/1
  bu/1 -> Sum1/3
  x1_dot/1 -> Sum1/2
  Sum1/1 -> Integrator/1
  Integrator/1 -> Sum/2  "x1_hat"
  x1/1 -> Sum/1

== system Y3Tiltrotor_sim3_IINDI_case2/Subsystem/多旋翼模态/Velocity Control/Improved INDI in vector form/6阶HOD ==
  X1 : Inport
  Gain : Gain  Gain=4*a_HOD_uvw^2.*eye(3)  Multiplication=Matrix(K*u) (u vector)
  Gain1 : Gain  Gain=4*a_HOD_uvw.*eye(3)  Multiplication=Matrix(K*u) (u vector)
  Integrator : Integrator  InitialCondition=[0 0 0]'
  Integrator1 : Integrator  InitialCondition=[0 0 0]'
  Sum : Sum  Inputs=|+-
  Sum1 : Sum  Inputs=++|
  X1_dot_hat : Outport
  wires:
  Gain1/1 -> Sum1/1
  Integrator1/1 -> Sum1/2  "x2_hat"
  Gain/1 -> Integrator1/1
  Sum1/1 -> Integrator/1, X1_dot_hat/1
  Sum/1 -> Gain1/1, Gain/1
  X1/1 -> Sum/1
  Integrator/1 -> Sum/2  "x1_hat"

== system Y3Tiltrotor_sim3_IINDI_case2/Subsystem/多旋翼模态/Velocity Control/Improved INDI in vector form/CFO ==
  x1_dot : Inport
  x1 : Inport  Port=2
  bu : Inport  Port=3
  Gain : Gain  Gain=[l_u 0 0;0 l_v 0;0 0 l_w]  Multiplication=Matrix(K*u) (u vector)
  Gain1 : Gain  Gain=[lamda_u 0 0;0 lamda_v 0;0 0 lamda_w]  Multiplication=Matrix(K*u) (u vector)
  Integrator : Integrator  InitialCondition=[0 0 0]'
  Integrator1 : Integrator  InitialCondition=[0 0 0]'
  Sum : Sum  Inputs=|+-
  Sum1 : Sum  Inputs=+++
  Sum2 : Sum  Inputs=++|
  d_hat : Outport
  wires:
  Sum2/1 -> d_hat/1, Sum1/1
  Integrator1/1 -> Sum2/2  "x2_hat"
  Gain1/1 -> Integrator1/1
  Sum/1 -> Gain/1
  Gain/1 -> Gain1/1, Sum2/1
  bu/1 -> Sum1/3
  x1_dot/1 -> Sum1/2
  Sum1/1 -> Integrator/1
  Integrator/1 -> Sum/2  "x1_hat"
  x1/1 -> Sum/1

== system Y3Tiltrotor_sim3_IINDI_case2/Subsystem/多旋翼模态/Velocity Control/Improved INDI in vector form/Subsystem3 ==
  original : Inport
  Demux : Demux  Outputs=3
  Mux : Mux  Inputs=3
  Transfer Fcn4 : TransferFcn  Numerator=[k_lpf_v]  Denominator=[1 k_lpf_v]
  Transfer Fcn5 : TransferFcn  Numerator=[k_lpf_w]  Denominator=[1 k_lpf_w]
  Transfer Fcn6 : TransferFcn  Numerator=[k_lpf_u]  Denominator=[1 k_lpf_u]
  LPF : Outport
  wires:
  Mux/1 -> LPF/1
  original/1 -> Demux/1
  Demux/2 -> Transfer Fcn4/1
  Transfer Fcn4/1 -> Mux/2
  Demux/3 -> Transfer Fcn5/1
  Transfer Fcn5/1 -> Mux/3
  Demux/1 -> Transfer Fcn6/1
  Transfer Fcn6/1 -> Mux/1

== system Y3Tiltrotor_sim3_IINDI_case2/Y3 Tiltrotor Aircraft Model/Subsystem/Aerodynamic Forces and Moments/Compute Body Frame Aerodynamic Forces and Moments/Aerodynamic Forces and Moment Calculations ==
  Coef_wind : Inport
  Q : Inport  Port=2
  AirData : Inport  Port=3
  Demux1 : Demux  Outputs=[3,3]
      settings: DisplayOption=none
  Mux : Mux  Inputs=3
  Product : Product  InputSameDT=on  OutDataTypeStr=Inherit: Inherit via back propagation  SaturateOnIntegerOverflow=on
  Product1 : Product  OutDataTypeStr=Inherit: Inherit via back propagation  SaturateOnIntegerOverflow=on
  Product3 : Product  InputSameDT=on  SaturateOnIntegerOverflow=on  OutDataTypeStr=Inherit: Same as first input
  Subsystem : Subsystem
  Subsystem1 : Subsystem  Commented=on
  b : Constant  Value=uavParam.geom.span
  cbar : Constant  Value=uavParam.geom.chord
  coefAdjust : Gain  Gain=[-1 1 -1]
  reference area : Gain  Gain=uavParam.geom.S  SaturateOnIntegerOverflow=on  OutDataTypeStr=Inherit: Same as input  ParamDataTypeStr=Inherit: Same as input
  Force_b : Outport
  Moment_b : Outport  Port=2
  wires:
  Mux/1 -> Product1/1
  cbar/1 -> Mux/2
  b/1 -> Mux/1, Mux/3
  Subsystem/1(F_b) -> Force_b/1
  Product/1 -> Subsystem/2(F_w)  "F_w"
  Demux1/1 -> coefAdjust/1
  Product1/1 -> Product3/2
  Demux1/2 -> Product3/1
  Coef_wind/1 -> Demux1/1
  Q/1 -> reference area/1
  reference area/1 -> Product1/2, Product/1
  coefAdjust/1 -> Product/2
  AirData/1 -> Subsystem/1(AirData)
  Product3/1 -> Moment_b/1  "M_w"

== system Y3Tiltrotor_sim3_IINDI_case2/Y3 Tiltrotor Aircraft Model/Subsystem/Aerodynamic Forces and Moments/Compute Body Frame Aerodynamic Forces and Moments/Wind frame F& M ==
  Airdata : Inport
  CtrlSurfaces : Inport  Port=2
  Bus Selector : BusSelector  OutputSignals=q
  Bus Selector3 : BusSelector  OutputSignals=dA1,dA2
  Bus Selector6 : BusSelector  OutputSignals=beta
  Bus Selector7 : BusSelector  OutputSignals=alpha
  Gain : Gain  Gain=1/2
  Gain1 : Gain  Gain=1/2
  Lateral Channel : Subsystem
  Longitudinal Channel : Subsystem
  Mux : Mux  Inputs=6
  Route coefficients : Subsystem
  Sum : Sum  Inputs=+-
  Sum1 : Sum
  coef : Outport  VectorParamsAs1DForOutWhenUnconnected=off
  Q : Outport  Port=2  VectorParamsAs1DForOutWhenUnconnected=off
  wires:
  Route coefficients/5(<Cm>) -> Mux/5  "Cm"
  Mux/1 -> coef/1
  Route coefficients/6(<Cn>) -> Mux/6  "Cn"
  Route coefficients/2(<CY>) -> Mux/2  "CY"
  Route coefficients/4(<Cl>) -> Mux/4  "Cl"
  Route coefficients/3(<CL>) -> Mux/3  "CL"
  Lateral Channel/1(Lateral) -> Route coefficients/1(Lateral)
  Longitudinal Channel/1(Longitudinal) -> Route coefficients/2(Longitudinal)
  Bus Selector7/1 -> Longitudinal Channel/1(alpha)  "<alpha>"
  Route coefficients/1(<CD>) -> Mux/1  "CD"
  Airdata/1 -> Bus Selector7/1, Bus Selector6/1, Bus Selector/1
  Bus Selector6/1 -> Lateral Channel/1(beta)  "<beta>"
  Bus Selector/1 -> Q/1  "<q>"
  CtrlSurfaces/1 -> Bus Selector3/1
  Gain/1 -> Longitudinal Channel/3(dA), Lateral Channel/2(dA)
  Gain1/1 -> Longitudinal Channel/2(dE)
  Sum/1 -> Gain/1
  Sum1/1 -> Gain1/1
  Bus Selector3/1 -> Sum1/2, Sum/1  "<dA1>"
  Bus Selector3/2 -> Sum1/1, Sum/2  "<dA2>"

== system Y3Tiltrotor_sim3_IINDI_case2/Y3 Tiltrotor Aircraft Model/Subsystem/GroundModel1/Ground Model New/If Action Subsystem ==
  mg3 : Inport
  ve3 : Inport  Port=2
  Action Port : ActionPort  ActionPortLabel=if(u1 < 0.05)
  Gain : Gain  Gain=-1
  Gain1 : Gain  Gain=-10
  Sum : Sum  Inputs=|++
  F13 : Outport  VectorParamsAs1DForOutWhenUnconnected=off
  wires:
  mg3/1 -> Gain/1
  ve3/1 -> Gain1/1
  Gain/1 -> Sum/1
  Gain1/1 -> Sum/2
  Sum/1 -> F13/1

== system Y3Tiltrotor_sim3_IINDI_case2/Y3 Tiltrotor Aircraft Model/Subsystem/GroundModel1/Ground Model New/If Action Subsystem1 ==
  mg3 : Inport
  ve3 : Inport  Port=2
  z : Inport  Port=3
  Action Port : ActionPort  ActionPortLabel=elseif(u1<0.1)
  Gain : Gain  Gain=-1
  Gain1 : Gain  Gain=-20
  Gain2 : Gain  Gain=-0.5
  Sum : Sum  Inputs=+++
  F13 : Outport  VectorParamsAs1DForOutWhenUnconnected=off
  wires:
  Gain1/1 -> Sum/2
  ve3/1 -> Gain1/1
  Sum/1 -> F13/1
  Gain/1 -> Sum/1
  mg3/1 -> Gain/1
  z/1 -> Gain2/1
  Gain2/1 -> Sum/3

== system Y3Tiltrotor_sim3_IINDI_case2/Y3 Tiltrotor Aircraft Model/Subsystem/GroundModel1/Ground Model New/If Action Subsystem2 ==
  mg3 : Inport
  ve3 : Inport  Port=2
  z : Inport  Port=3
  Action Port : ActionPort  ActionPortLabel=else
  Gain : Gain  Gain=-1
  Gain1 : Gain  Gain=-50
  Gain2 : Gain  Gain=-1
  Sum : Sum  Inputs=+++
  F13 : Outport  VectorParamsAs1DForOutWhenUnconnected=off
  wires:
  mg3/1 -> Gain/1
  ve3/1 -> Gain1/1
  Gain1/1 -> Sum/2
  Gain/1 -> Sum/1
  Gain2/1 -> Sum/3
  Sum/1 -> F13/1
  z/1 -> Gain2/1

== system Y3Tiltrotor_sim3_IINDI_case2/Y3 Tiltrotor Aircraft Model/Subsystem/Propulsion/Rotor Assembly 1/Adjust Force to Body Frame ==
  note: 考虑旋翼桨叶的挥舞运动时，旋翼的旋转方向会影响桨毂坐标系下y轴的受力
  Fmotor : Inport
  Tilt : Inport  Port=2
  TurnDirection : Inport  Port=3
  Constant : Constant
  Constant1 : Constant
  Constant2 : Constant  Value=0
  Constant3 : Constant  Value=0
  Coordinate Transformation Conversion : robotcorelib/Coordinate Transformation Conversion  InputRepresentation=Euler Angles  InputEulerSequence=ZYX  ShowTrVecInputPort=on  OutputRepresentation=Rotation Matrix  OutputEulerSequence=ZYX  ShowTrVecOutputPort=on  SimulateUsing=Code generation
      settings: LibrarySourceBlock=uavutilslib/Coordinate Transformation Conversion
  Gain2 : Gain  Gain=-1
  Mux : Mux  Inputs=3
  Mux1 : Mux  Inputs=3
  Product : Product
  Product2 : Product  Multiplication=Matrix(*)
  Fbody : Outport
  wires:
  Constant1/1 -> Mux/3
  Constant/1 -> Mux/1
  Constant3/1 -> Mux1/3
  Constant2/1 -> Mux1/1
  Product2/1 -> Fbody/1
  Coordinate Transformation Conversion/1 -> Product2/1
  Mux/1 -> Product/2
  Product/1 -> Product2/2
  Gain2/1 -> Mux1/2
  TurnDirection/1 -> Mux/2
  Mux1/1 -> Coordinate Transformation Conversion/1
  Tilt/1 -> Gain2/1
  Fmotor/1 -> Product/1

== system Y3Tiltrotor_sim3_IINDI_case2/Y3 Tiltrotor Aircraft Model/Subsystem/Propulsion/Rotor Assembly 2/Adjust Force to Body Frame ==
  Fmotor : Inport
  Tilt : Inport  Port=2
  TurnDirection : Inport  Port=3
  Constant : Constant
  Constant1 : Constant
  Constant2 : Constant  Value=0
  Constant3 : Constant  Value=0
  Coordinate Transformation Conversion : robotcorelib/Coordinate Transformation Conversion  InputRepresentation=Euler Angles  InputEulerSequence=ZYX  ShowTrVecInputPort=on  OutputRepresentation=Rotation Matrix  OutputEulerSequence=ZYX  ShowTrVecOutputPort=on  SimulateUsing=Code generation
      settings: LibrarySourceBlock=uavutilslib/Coordinate Transformation Conversion
  Gain2 : Gain  Gain=-1
  Mux : Mux  Inputs=3
  Mux1 : Mux  Inputs=3
  Product : Product
  Product2 : Product  Multiplication=Matrix(*)
  Fbody : Outport
  wires:
  Mux1/1 -> Coordinate Transformation Conversion/1
  TurnDirection/1 -> Mux/2
  Gain2/1 -> Mux1/2
  Product/1 -> Product2/2
  Mux/1 -> Product/2
  Coordinate Transformation Conversion/1 -> Product2/1
  Product2/1 -> Fbody/1
  Constant2/1 -> Mux1/1
  Constant3/1 -> Mux1/3
  Constant/1 -> Mux/1
  Constant1/1 -> Mux/3
  Fmotor/1 -> Product/1
  Tilt/1 -> Gain2/1

== system Y3Tiltrotor_sim3_IINDI_case2/Y3 Tiltrotor Aircraft Model/Subsystem/Propulsion/Rotor Assembly 3 /Adjust Force to Body Frame ==
  Fmotor : Inport
  Tilt : Inport  Port=2
  TurnDirection : Inport  Port=3
  Constant : Constant
  Constant1 : Constant
  Constant2 : Constant  Value=0
  Constant4 : Constant  Value=0
  Coordinate Transformation Conversion : robotcorelib/Coordinate Transformation Conversion  InputRepresentation=Euler Angles  InputEulerSequence=ZYX  ShowTrVecInputPort=on  OutputRepresentation=Rotation Matrix  OutputEulerSequence=ZYX  ShowTrVecOutputPort=on  SimulateUsing=Code generation
      settings: LibrarySourceBlock=uavutilslib/Coordinate Transformation Conversion
  Gain2 : Gain  Gain=-1
  Mux : Mux  Inputs=3
  Mux1 : Mux  Inputs=3
  Product : Product
  Product2 : Product  Multiplication=Matrix(*)
  Fbody : Outport
  wires:
  Constant1/1 -> Mux/3
  Constant/1 -> Mux/1
  Constant2/1 -> Mux1/1
  Product2/1 -> Fbody/1
  Coordinate Transformation Conversion/1 -> Product2/1
  Mux/1 -> Product/2
  Product/1 -> Product2/2
  TurnDirection/1 -> Mux/2
  Mux1/1 -> Coordinate Transformation Conversion/1
  Fmotor/1 -> Product/1
  Tilt/1 -> Gain2/1
  Gain2/1 -> Mux1/3
  Constant4/1 -> Mux1/2

== system Y3Tiltrotor_sim3_IINDI_case2/Y3 Tiltrotor Aircraft Model/Subsystem/Weather Model_org/[0, pi] Wrap Around/Negative Yaw ==
  yaw : Inport
  Enable : EnablePort
  Abs : Abs  SaturateOnIntegerOverflow=off
  Constant1 : Constant  Value=2*pi
      settings: AttributesFormatString=%<Value>
  Constant2 : Constant  Value=2*pi
      settings: AttributesFormatString=%<Value>
  Math Function : Math  Operator=mod  SignedPower=on
  Sum : Sum  Inputs=|-+
  yaw_wr : Outport  VectorParamsAs1DForOutWhenUnconnected=off
  wires:
  Sum/1 -> yaw_wr/1
  Constant2/1 -> Sum/2
  Abs/1 -> Math Function/1
  Math Function/1 -> Sum/1
  Constant1/1 -> Math Function/2
  yaw/1 -> Abs/1

== system Y3Tiltrotor_sim3_IINDI_case2/Y3 Tiltrotor Aircraft Model/Subsystem/Weather Model_org/[0, pi] Wrap Around/Positive Yaw ==
  yaw : Inport
  Enable : EnablePort
  Constant1 : Constant  Value=2*pi
      settings: AttributesFormatString=%<Value>
  Math Function : Math  Operator=mod  SignedPower=on
  yaw_wr : Outport  VectorParamsAs1DForOutWhenUnconnected=off
  wires:
  Math Function/1 -> yaw_wr/1
  Constant1/1 -> Math Function/2
  yaw/1 -> Math Function/1

== system Y3Tiltrotor_sim3_IINDI_case2/Subsystem/固定翼模态/高度-速度控制/定速模式/Subsystem1/Subsystem ==
  Manual : Inport
  Height_d : Inport  Port=2
  Manual Vz_d : Inport  Port=3
  Xe : Inport  Port=4
  InputConditioning_altitude : Subsystem
  Merge : Merge
  Subsystem : Subsystem
  Switch Case : SwitchCase  CaseConditions={0,1}  ShowDefaultCase=off
  Vz_d : Outport
  wires:
  Manual/1 -> Switch Case/1
  Xe/1 -> Subsystem/2(Xe), InputConditioning_altitude/2(Xe)
  Subsystem/1(PID_vz_cmd) -> Merge/1  "PID vz_d"
  InputConditioning_altitude/1(manual_vz_cmd) -> Merge/2  "Manual vz_d"
  Merge/1 -> Vz_d/1
  Switch Case/1 -> Subsystem/Action
  Switch Case/2 -> InputConditioning_altitude/Action
  Manual Vz_d/1 -> InputConditioning_altitude/1(Manual Vz_d)
  Height_d/1 -> Subsystem/1(Navigation Z)

== system Y3Tiltrotor_sim3_IINDI_case2/Subsystem/固定翼模态/高度-速度控制/定高模式/Subsystem/InputConditioning_altitude ==
  Manual Vz_d : Inport
  Xe : Inport  Port=2
  Action Port : ActionPort  ActionPortLabel=case [ 1 ]:
  MATLAB Function : MATLAB Function  TreatAsAtomicUnit=on
  Selector : Selector  InputPortWidth=3  IndexOptions=Index vector (dialog)  Indices=3  OutputSizes=1
  manual_vz_cmd : Outport  VectorParamsAs1DForOutWhenUnconnected=off
  wires:
  MATLAB Function/1(vz_cmd) -> manual_vz_cmd/1
  Manual Vz_d/1 -> MATLAB Function/1(u)
  Selector/1 -> MATLAB Function/2(z_e)
  Xe/1 -> Selector/1

== system Y3Tiltrotor_sim3_IINDI_case2/Subsystem/固定翼模态/高度-速度控制/定高模式/Subsystem/Subsystem ==
  Navigation Z : Inport
  Xe : Inport  Port=2
  Action Port : ActionPort  ActionPortLabel=case [ 0 ]:
  PID Controller1 : slpidlib/PID Controller  Controller=PID  Form=Parallel  TimeDomain=Continuous-time  UseExternalTs=off  SampleTime=ControlSampleTime  IntegratorMethod=Forward Euler  FilterMethod=Forward Euler  ControllerParametersSource=internal  P=control.FW.alt_P  I=control.FW.alt_I  UseKiTs=off  D=control.FW.alt_D  UseExternalDerivativeSource=off  N=100  UseFilter=on  TunerSelectOption=Transfer Function Based (PID Tuner App)  InitialConditionSource=internal  InitialConditionForIntegrator=0  InitialConditionForFilter=0  DifferentiatorICPrevScaledInput=0  ExternalReset=none  TrackingMode=off  Kt=1  LimitOutput=on  SatLimitsSource=internal  UpperSaturationLimit=control.maxClimbRate  LowerSaturationLimit=control.maxDescendRate  LinearizeAsGain=on  AntiWindupMode=clamping  Kb=1  LimitIntegrator=off  UpperIntegratorSaturationLimit=inf  LowerIntegratorSaturationLimit=-inf  POutMin=[]  POutMax=[]  IOutMin=[]  IOutMax=[]  DOutMin=[]  DOutMax=[]  NOutMin=[]  NOutMax=[]  SumOutMin=[]  SumOutMax=[]  SaturationOutMin=[]  SaturationOutMax=[]  PParamMin=[]  PParamMax=[]  IParamMin=[]  IParamMax=[]  DParamMin=[]  DParamMax=[]  NParamMin=[]  NParamMax=[]  KbParamMin=[]  KbParamMax=[]  KtParamMin=[]  KtParamMax=[]  KbOutMin=[]  KbOutMax=[]  KtOutMin=[]  KtOutMax=[]  IntegratorOutMin=[]  IntegratorOutMax=[]  FilterOutMin=[]  FilterOutMax=[]  SumI1OutMin=[]  SumI1OutMax=[]  SumI2OutMin=[]  SumI2OutMax=[]  SumI3OutMin=[]  SumI3OutMax=[]  SumI4OutMin=[]  SumI4OutMax=[]  SumDOutMin=[]  SumDOutMax=[]  DifferentiatorOutMin=[]  DifferentiatorOutMax=[]  FilterDiffOutCoefMin=[]  FilterDiffOutCoefMax=[]  ReciprocalOutMin=[]  ReciprocalOutMax=[]  SumDenOutMin=[]  SumDenOutMax=[]  SumNumOutMin=[]  SumNumOutMax=[]  DivideOutMin=[]  DivideOutMax=[]  UdiffTsProdOutMin=[]  UdiffTsProdOutMax=[]  NTsProdOutMin=[]  NTsProdOutMax=[]  UintegralTsProdOutMin=[]  UintegralTsProdOutMax=[]  UngainTsProdOutMin=[]  UngainTsProdOutMax=[]  ClampingZeroOutDataTypeStr=Inherit: Inherit via back propagation  ClampingZeroOutMin=[]  ClampingZeroOutMax=[]  FilterDenConstantOutDataTypeStr=Inherit: Inherit via back propagation  FilterDenConstantOutMin=[]  FilterDenConstantOutMax=[]  PCopyOutDataTypeStr=Inherit: Inherit via back propagation  PCopyOutMin=[]  PCopyOutMax=[]  NCopyOutDataTypeStr=Inherit: Inherit via back propagation  NCopyOutMin=[]  NCopyOutMax=[]  IntegratorContinuousStateAttributes=''  IntegratorStateMustResolveToSignalObject=off  IntegratorRTWStateStorageClass=Auto  FilterContinuousStateAttributes=''  FilterStateMustResolveToSignalObject=off  FilterRTWStateStorageClass=Auto  ParallelPVariant=InternalParameters  IdealPVariant=Disabled  IVariant=InternalParameters  DVariant=InternalParameters  IntegratorVariant=Continuous  SatVariant=Enabled  AWVariant=ContClampingParallel  PCopyVariant=Disabled  TRVariant=Disabled  FdbkBlocksVariant=Forward  IdealPFdbkVariant=Disabled  SatFdbkVariant=Disabled  DerivativeFilterVariant=ContFilter  NVariant=InternalParameters  NCopyVariant=Disabled  FilterICVariant=InternalICsFilter  IntegratorICVariant=InternalICs  ExternalResetVariant=Disabled  TRSumVariant=Passthrough  SumFdbkVariant=Disabled  SumVariant=Sum_PID  TsampFilterVariant=InternalTs  TsampNgainVariant=Passthrough  TsampIntegralVariant=Disabled_SignalSpec  ExternalSaturationOutDataTypeStr=Inherit: Same as second input  DerivativeSourceVariant=ErrorSignal  PreIntVariant=InternalPreInt
  Selector : Selector  InputPortWidth=3  IndexOptions=Index vector (dialog)  Indices=3  OutputSizes=1
  Sum : Sum  Inputs=|+-
  Unary Minus : UnaryMinus
  PID_vz_cmd : Outport
  wires:
  Unary Minus/1 -> Sum/2
  Selector/1 -> Unary Minus/1
  Xe/1 -> Selector/1
  Sum/1 -> PID Controller1/1
  PID Controller1/1 -> PID_vz_cmd/1
  Navigation Z/1 -> Sum/1

== system Y3Tiltrotor_sim3_IINDI_case2/Y3 Tiltrotor Aircraft Model/Subsystem/Aerodynamic Forces and Moments/Compute Body Frame Aerodynamic Forces and Moments/Aerodynamic Forces and Moment Calculations/Subsystem ==
  AirData : Inport
  F_w : Inport  Port=2
  Bus Selector : BusSelector  OutputSignals=alpha,beta
  Direction Cosine Matrix Body to Wind : aerolibtransform2/Direction Cosine Matrix Body to Wind
  Mux1 : Mux  Inputs=2
  Product2 : Product  Multiplication=Matrix(*)  RndMeth=Zero
  Reshape1 : Reshape  OutputDimensionality=Column vector (2-D)
  Reshape2 : Reshape
  Transpose : Math  Operator=transpose  SignedPower=on
  F_b : Outport
  wires:
  Transpose/1 -> Product2/1
  Product2/1 -> Reshape2/1
  Mux1/1 -> Direction Cosine Matrix Body to Wind/1
  F_w/1 -> Reshape1/1
  Reshape1/1 -> Product2/2
  Reshape2/1 -> F_b/1
  Direction Cosine Matrix Body to Wind/1 -> Transpose/1
  Bus Selector/1 -> Mux1/1  "<alpha>"
  Bus Selector/2 -> Mux1/2  "<beta>"
  AirData/1 -> Bus Selector/1

== system Y3Tiltrotor_sim3_IINDI_case2/Y3 Tiltrotor Aircraft Model/Subsystem/Aerodynamic Forces and Moments/Compute Body Frame Aerodynamic Forces and Moments/Aerodynamic Forces and Moment Calculations/Subsystem1 ==
  AirData : Inport
  M_w : Inport  Port=2
  Bus Selector : BusSelector  OutputSignals=alpha,beta
  Direction Cosine Matrix Body to Wind : aerolibtransform2/Direction Cosine Matrix Body to Wind
  Mux1 : Mux  Inputs=2
  Product2 : Product  Multiplication=Matrix(*)  RndMeth=Zero
  Reshape1 : Reshape  OutputDimensionality=Column vector (2-D)
  Reshape2 : Reshape
  Transpose : Math  Operator=transpose  SignedPower=on
  M_b : Outport
  wires:
  AirData/1 -> Bus Selector/1
  Bus Selector/2 -> Mux1/2  "<beta>"
  Bus Selector/1 -> Mux1/1  "<alpha>"
  Direction Cosine Matrix Body to Wind/1 -> Transpose/1
  Reshape2/1 -> M_b/1
  Reshape1/1 -> Product2/2
  M_w/1 -> Reshape1/1
  Mux1/1 -> Direction Cosine Matrix Body to Wind/1
  Product2/1 -> Reshape2/1
  Transpose/1 -> Product2/1
